simulink model "ex2_sim"  (R2023b)
settings: Solver=FixedStepAuto  StartTime=0.0  StopTime=30  FixedStep=0.0001  RelTol=1e-3
InitFcn:
  | ex2
values from neighbouring files (symbols this model uses):
  N0 = 8    [ex1.m]    (also in ex2.m = 4)
  Nq = [(1 - 0.1) / (1 + 0.1), (1 - 0.2) / (1 + 0.2)]'    [ex1.m]    (also in ex2.m = [(1 - 0.26) / (1 + 0.26), (1 - 0.15) / (1 + 0.15), (1 - 0.17)
undefined symbols (not defined in the file or in its folder): A, B, C, D, F, F_A, F_B, F_E, F_F
libraries: simulink x7
settings Model: Creator=赵生  LastModifiedBy=赵生
settings OptimizationCC: DefaultParameterBehavior=Inlined  EnhancedBackFolding=on  PassReuseOutputArgsAs=Individual arguments  ZeroExternalMemoryAtStartup=off  ZeroInternalMemoryAtStartup=off  OptimizeBlockOrder=speed  DifferentSizesBufferReuse=on  OptimizationCustomize=off  EfficientTunableParamExpr=on
settings DebuggingCC: ParameterTunabilityLossMsg=error
settings SFSimCC: MATLABDynamicMemAlloc=off
settings RTWCC: Description=Embedded Coder  SystemTargetFile=ert.tlc  TemplateMakefile=ert_default_tmf
settings CodeAppCC: ForceParamTrailComments=on  IgnoreCustomStorageClasses=off  OperatorAnnotations=on  SimulinkDataObjDesc=on  SFDataObjDesc=on  InsertBlockDesc=on
settings ERTTargetCC: TargetLangStandard=C99 (ISO)  GenerateSampleERTMain=on  SupportContinuousTime=on  InlinedParameterPlacement=NonHierarchical  ERTCustomFileTemplate=example_file_process.tlc

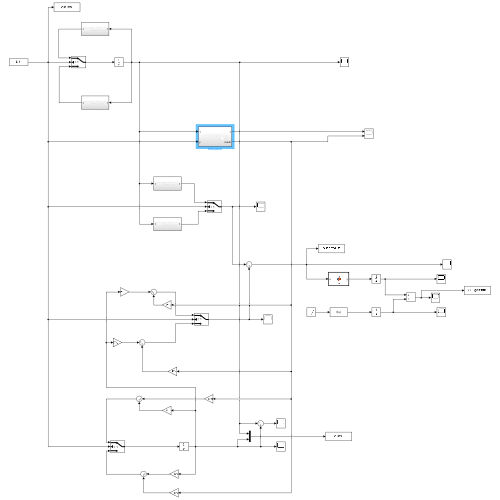
[thumbnail: Simulink's stored preview of the top-level diagram]
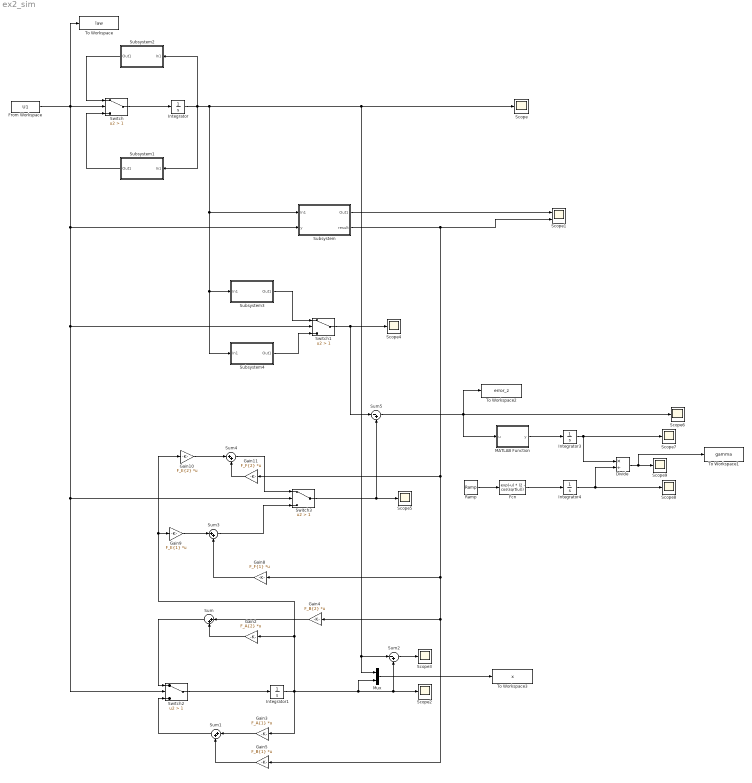
== system ex2_sim ==
  Divide : Product  Inputs=*/
  Fcn : Fcn  Expr=exp(-u) * (2 - cos(sqrt(u)))
  From Workspace : FromWorkspace  VariableName=U1
  Gain10 : Gain  Gain=F_E{2}  Multiplication=Matrix(K*u)
  Gain11 : Gain  Gain=F_F{2}  Multiplication=Matrix(K*u)
  Gain2 : Gain  Gain=F_A{2}  Multiplication=Matrix(K*u)
  Gain3 : Gain  Gain=F_A{1}  Multiplication=Matrix(K*u)
  Gain4 : Gain  Gain=F_B{2}  Multiplication=Matrix(K*u)
  Gain5 : Gain  Gain=F_B{1}  Multiplication=Matrix(K*u)
  Gain8 : Gain  Gain=F_F{1}  Multiplication=Matrix(K*u)
  Gain9 : Gain  Gain=F_E{1}  Multiplication=Matrix(K*u)
  Integrator : Integrator  InitialCondition=[0 0 0]'
  Integrator1 : Integrator  InitialCondition=[0 0 0]'
  Integrator3 : Integrator
  Integrator4 : Integrator
  MATLAB Function : MATLAB Function  TreatAsAtomicUnit=on
  Mux : Mux  Inputs=2
  Ramp : simulink/Sources/Ramp  slope=1  start=0  InitialOutput=0
  Scope{,2..9} (9 alike) : Scope
  Scope1 : Scope  NumInputPorts=2
  Subsystem : Subsystem
  Subsystem1 : Subsystem
  Subsystem2 : Subsystem
  Subsystem3 : Subsystem
  Subsystem4 : Subsystem
  Sum{,1,3..4} (4 alike) : Sum  Inputs=|++
  Sum2 : Sum  Inputs=|-+
  Sum5 : Sum  Inputs=|-+
  Switch{,1..3} (4 alike) : Switch  Criteria=u2 > Threshold  Threshold=1  SaturateOnIntegerOverflow=off  InputSameDT=off
  To Workspace : ToWorkspace  VariableName=law  SaveFormat=Structure With Time  SampleTime=-1
  To Workspace1 : ToWorkspace  VariableName=gamma  SaveFormat=Structure With Time  SampleTime=-1
  To Workspace2 : ToWorkspace  VariableName=error_z  SaveFormat=Structure With Time  SampleTime=-1
  To Workspace3 : ToWorkspace  VariableName=x  SaveFormat=Structure With Time  SampleTime=-1
  wires:
  Sum3/1 -> Switch3/3
  Subsystem/2(result) -> Scope1/2, Gain11/1, Gain8/1, Gain4/1, Gain5/1
  Subsystem3/1(Out1) -> Switch1/1
  Switch1/1 -> Sum5/1, Scope4/1
  From Workspace/1 -> To Workspace/1, Switch2/2, Switch3/2, Switch1/2, Subsystem/2(y), Switch/2
  Gain3/1 -> Sum1/1
  Gain9/1 -> Sum3/1
  Sum/1 -> Switch2/1
  Gain8/1 -> Sum3/2
  Gain5/1 -> Sum1/2
  Subsystem2/1(Out1) -> Switch/1
  Sum2/1 -> Scope3/1
  Integrator/1 -> Scope/1, Mux/1, Sum2/1, Subsystem/1(In1), Subsystem4/1(In1), Subsystem3/1(In1), Subsystem2/1(In1), Subsystem1/1(In1)
  Switch2/1 -> Integrator1/1
  Integrator1/1 -> Gain9/1, Gain10/1, Gain2/1, Mux/2, Sum2/2, Scope2/1, Gain3/1
  Subsystem/1(Out1) -> Scope1/1
  Sum1/1 -> Switch2/3
  Gain10/1 -> Sum4/1
  Sum4/1 -> Switch3/1
  Gain4/1 -> Sum/1
  Subsystem4/1(Out1) -> Switch1/3
  Gain11/1 -> Sum4/2
  Switch3/1 -> Scope5/1, Sum5/2
  Gain2/1 -> Sum/2
  Sum5/1 -> To Workspace2/1, MATLAB Function/1(u), Scope6/1
  Switch/1 -> Integrator/1
  Subsystem1/1(Out1) -> Switch/3
  Ramp/1 -> Fcn/1
  Divide/1 -> To Workspace1/1, Scope9/1
  MATLAB Function/1(y) -> Integrator3/1
  Integrator3/1 -> Divide/1, Scope7/1
  Fcn/1 -> Integrator4/1
  Integrator4/1 -> Divide/2, Scope8/1
  Mux/1 -> To Workspace3/1

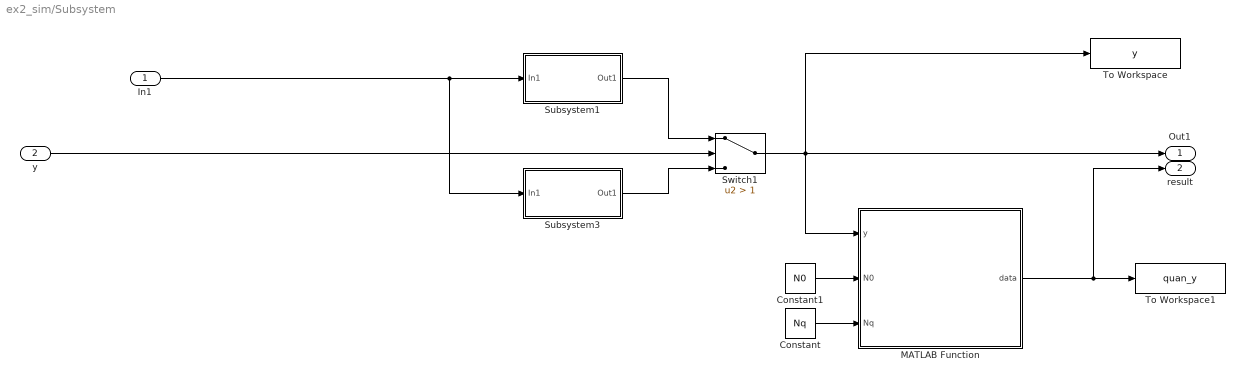
== system ex2_sim/Subsystem ==
  In1 : Inport
  y : Inport  Port=2
  Constant : Constant  Value=Nq
  Constant1 : Constant  Value=N0
  MATLAB Function : MATLAB Function  TreatAsAtomicUnit=on
  Subsystem1 : Subsystem
  Subsystem3 : Subsystem
  Switch1 : Switch  Criteria=u2 > Threshold  Threshold=1  SaturateOnIntegerOverflow=off  InputSameDT=off
  To Workspace : ToWorkspace  VariableName=y  SaveFormat=Structure With Time  SampleTime=-1
  To Workspace1 : ToWorkspace  VariableName=quan_y  SaveFormat=Structure With Time  SampleTime=-1
  Out1 : Outport
  result : Outport  Port=2
  wires:
  Switch1/1 -> Out1/1, To Workspace/1, MATLAB Function/1(y)
  MATLAB Function/1(data) -> result/1, To Workspace1/1
  Subsystem3/1(Out1) -> Switch1/3
  In1/1 -> Subsystem3/1(In1), Subsystem1/1(In1)
  Constant/1 -> MATLAB Function/3(Nq)
  Subsystem1/1(Out1) -> Switch1/1
  Constant1/1 -> MATLAB Function/2(N0)
  y/1 -> Switch1/2

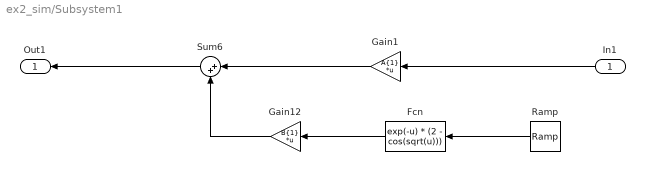
== system ex2_sim/Subsystem1 ==
  In1 : Inport
  Fcn : Fcn  Expr=exp(-u) * (2 - cos(sqrt(u)))
  Gain1 : Gain  Gain=A{1}  Multiplication=Matrix(K*u)
  Gain12 : Gain  Gain=B{1}  Multiplication=Matrix(K*u)
  Ramp : simulink/Sources/Ramp  slope=1  start=0  InitialOutput=0
  Sum6 : Sum  Inputs=|++
  Out1 : Outport
  wires:
  Sum6/1 -> Out1/1
  Gain1/1 -> Sum6/1
  Ramp/1 -> Fcn/1
  Gain12/1 -> Sum6/2
  Fcn/1 -> Gain12/1
  In1/1 -> Gain1/1

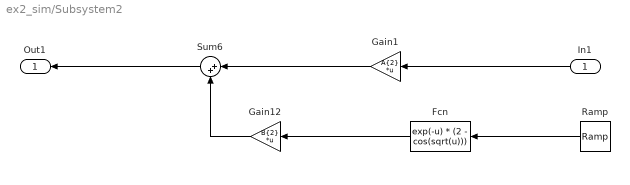
== system ex2_sim/Subsystem2 ==
  In1 : Inport
  Fcn : Fcn  Expr=exp(-u) * (2 - cos(sqrt(u)))
  Gain1 : Gain  Gain=A{2}  Multiplication=Matrix(K*u)
  Gain12 : Gain  Gain=B{2}  Multiplication=Matrix(K*u)
  Ramp : simulink/Sources/Ramp  slope=1  start=0  InitialOutput=0
  Sum6 : Sum  Inputs=|++
  Out1 : Outport
  wires:
  Sum6/1 -> Out1/1
  Gain1/1 -> Sum6/1
  Ramp/1 -> Fcn/1
  Gain12/1 -> Sum6/2
  Fcn/1 -> Gain12/1
  In1/1 -> Gain1/1

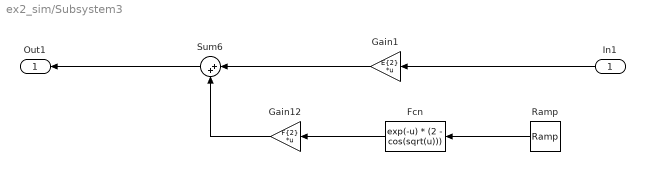
== system ex2_sim/Subsystem3 ==
  In1 : Inport
  Fcn : Fcn  Expr=exp(-u) * (2 - cos(sqrt(u)))
  Gain1 : Gain  Gain=E{2}  Multiplication=Matrix(K*u)
  Gain12 : Gain  Gain=F{2}  Multiplication=Matrix(K*u)
  Ramp : simulink/Sources/Ramp  slope=1  start=0  InitialOutput=0
  Sum6 : Sum  Inputs=|++
  Out1 : Outport
  wires:
  Sum6/1 -> Out1/1
  Gain1/1 -> Sum6/1
  Ramp/1 -> Fcn/1
  Gain12/1 -> Sum6/2
  Fcn/1 -> Gain12/1
  In1/1 -> Gain1/1

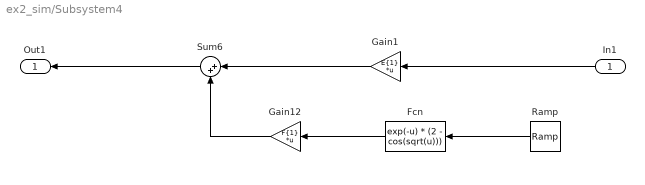
== system ex2_sim/Subsystem4 ==
  In1 : Inport
  Fcn : Fcn  Expr=exp(-u) * (2 - cos(sqrt(u)))
  Gain1 : Gain  Gain=E{1}  Multiplication=Matrix(K*u)
  Gain12 : Gain  Gain=F{1}  Multiplication=Matrix(K*u)
  Ramp : simulink/Sources/Ramp  slope=1  start=0  InitialOutput=0
  Sum6 : Sum  Inputs=|++
  Out1 : Outport
  wires:
  Sum6/1 -> Out1/1
  Gain1/1 -> Sum6/1
  Ramp/1 -> Fcn/1
  Gain12/1 -> Sum6/2
  Fcn/1 -> Gain12/1
  In1/1 -> Gain1/1

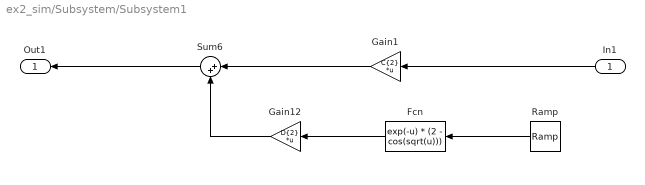
== system ex2_sim/Subsystem/Subsystem1 ==
  In1 : Inport
  Fcn : Fcn  Expr=exp(-u) * (2 - cos(sqrt(u)))
  Gain1 : Gain  Gain=C{2}  Multiplication=Matrix(K*u)
  Gain12 : Gain  Gain=D{2}  Multiplication=Matrix(K*u)
  Ramp : simulink/Sources/Ramp  slope=1  start=0  InitialOutput=0
  Sum6 : Sum  Inputs=|++
  Out1 : Outport
  wires:
  Sum6/1 -> Out1/1
  Gain1/1 -> Sum6/1
  Ramp/1 -> Fcn/1
  Gain12/1 -> Sum6/2
  Fcn/1 -> Gain12/1
  In1/1 -> Gain1/1

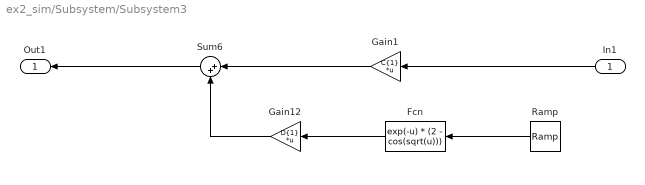
== system ex2_sim/Subsystem/Subsystem3 ==
  In1 : Inport
  Fcn : Fcn  Expr=exp(-u) * (2 - cos(sqrt(u)))
  Gain1 : Gain  Gain=C{1}  Multiplication=Matrix(K*u)
  Gain12 : Gain  Gain=D{1}  Multiplication=Matrix(K*u)
  Ramp : simulink/Sources/Ramp  slope=1  start=0  InitialOutput=0
  Sum6 : Sum  Inputs=|++
  Out1 : Outport
  wires:
  Sum6/1 -> Out1/1
  Gain1/1 -> Sum6/1
  Ramp/1 -> Fcn/1
  Gain12/1 -> Sum6/2
  Fcn/1 -> Gain12/1
  In1/1 -> Gain1/1

== matlab function ex2_sim/Subsystem/MATLAB Function ==
  data: y input; N0 input; data output; Nq input
function data = quantize_2d(y, N0, Nq)
data = zeros(size(y));
for c = 1:3
    yc = y(c, :);
    aleph = Nq(c);
    psi0 = N0;
    idx = yc > 0;
    if any(idx) 
        phi = ceil(log(yc(idx) / (psi0 * (1 + aleph) / 2)) / log(aleph));
        data(c, idx) = (aleph.^phi) * psi0;
    end
end

== matlab function ex2_sim/MATLAB Function ==
  data: u input; y output
function y = fcn(u)

y = [1 1 1] * u ;
